simulink model "tractor_mu1109"  (R2022b)
settings: Solver=FixedStepDiscrete  StartTime=0.0  StopTime=20  FixedStep=0.001  RelTol=1e-3
model workspace (MAT data in the model file):
  P : object (value not decoded)
  w_2 : Simulink.Parameter (value not decoded)
undefined symbols (not defined in the file): A, a, B, b, C, D, DiscIntNeverNeededParam, Iz, K, k1, K1, k2, K2, L1, L2, m, magnitude, Phi, Sample_time, Steer_Ratio
libraries: simulink x26, slpidlib x13, Solver_SF x1, dsparch4 x1
(part 7 of 7)

== matlab function tractor_mu1109/软土扭矩分配/CBF-QP扭矩分配 ==
  data: dt_s input; selected_torques_n_m output; kappa input; dot_kappa input; kappa_valid input; input_gains input; previous_applied_torques_n_m input; nominal_torques_n_m input; base_torques_n_m input; wheel_limits_n_m input; front_steers_rad input; total_torque_n_m input; control_mz_n_m input; cbf_torque_upper_bounds output; cbf_active output; qp_status output; qp_objective output; disturbance_state_out output; disturbance_margins output
function [selected_torques_n_m, cbf_torque_upper_bounds, cbf_active, qp_status, qp_objective, disturbance_state_out, disturbance_margins] = MF_CBF_QP_TorqueAllocator(dt_s, kappa, dot_kappa, kappa_valid, input_gains, previous_applied_torques_n_m, nominal_torques_n_m, base_torques_n_m, wheel_limits_n_m, front_steers_rad, total_torque_n_m, control_mz_n_m)

% CBF-QP 安全扭矩分配模块
%
% 本模块完成：
% 1）滑移率动力学扰动估计；
% 2）CBF滑移安全扭矩上界计算；
% 3）考虑前轮转角的横摆力矩系数计算；
% 4）四轮扭矩QP优化分配。

persistent disturbance_state

if isempty(disturbance_state)
    disturbance_state = zeros(1, 4);
end

%% 输入整理

dt = max(double(dt_s), 0.0);

kappa_vec = row4_local(kappa);
dot_kappa_vec = row4_local(dot_kappa);
valid_vec = row4_local(kappa_valid);
gain_vec = row4_local(input_gains);
applied_vec = row4_local(previous_applied_torques_n_m);
nominal_vec = row4_local(nominal_torques_n_m);
base_vec = row4_local(base_torques_n_m);
limit_vec = row4_local(wheel_limits_n_m);

total_target = double(total_torque_n_m);
yaw_target = double(control_mz_n_m);

steer_input = double(front_steers_rad);

if numel(steer_input) >= 2
    delta_l = steer_input(1);
    delta_r = steer_input(2);
else
    delta_l = steer_input(1);
    delta_r = steer_input(1);
end

%% 轮端限幅整理

wheel_limits = zeros(1, 4);
base_torques = zeros(1, 4);
nominal_torques = zeros(1, 4);

for index = 1:4

    wheel_limits(index) = max(0.0, limit_vec(index));

    base_torques(index) = clamp_local(base_vec(index), 0.0, wheel_limits(index));

    nominal_torques(index) = clamp_local(nominal_vec(index), 0.0, wheel_limits(index));
end

%% 一、等效扰动估计

% 滑移率动力学：
% dot(kappa_i) = g_i * T_i + d_i
%
% 等效扰动估计：
% d_i = dot(kappa_i) - g_i * T_i

disturbance_margins = zeros(1, 4);
alpha_disturbance = first_order_alpha_local(dt, 0.15);

for index = 1:4

    gain = gain_vec(index);

    if valid_vec(index) > 0.5 && isfinite(gain)

        raw_estimate = dot_kappa_vec(index) - gain * applied_vec(index);

        disturbance_state(index) = disturbance_state(index) + ...
            alpha_disturbance * (raw_estimate - disturbance_state(index));

        residual = raw_estimate - disturbance_state(index);

    else

        residual = 0.0;
    end

    % 扰动估计不确定性裕度。
    disturbance_margins(index) = clamp_local(0.05 + 0.05 * abs(residual), 0.05, 5.0);
end

disturbance_state_out = disturbance_state;

%% 二、CBF滑移安全扭矩上界计算

% 安全函数：
% h_i = kappa_max - kappa_i
%
% CBF条件：
% dot(h_i) + gamma*h_i >= 0
%
% 由 dot(kappa_i) = g_i*T_i + d_i 可得：
% g_i*T_i + d_i + margin_i <= gamma*(kappa_max - kappa_i)
%
% 因此：
% T_i <= [gamma*(kappa_max-kappa_i) - d_i - margin_i] / g_i

kappa_max = 0.25;
cbf_gamma = 15.0;

cbf_torque_upper_bounds = zeros(1, 4);
cbf_active = zeros(1, 4);

for index = 1:4

    gain = gain_vec(index);

    if valid_vec(index) > 0.5 && isfinite(gain) && isfinite(kappa_vec(index))

        upper = (cbf_gamma * (kappa_max - kappa_vec(index)) ...
            - disturbance_state(index) ...
            - disturbance_margins(index)) / gain;

        if ~isfinite(upper)
            upper = wheel_limits(index);
        end

        upper = clamp_local(upper, 0.0, wheel_limits(index));

    else

        upper = wheel_limits(index);
    end

    cbf_torque_upper_bounds(index) = upper;

    % 若CBF上界低于基线扭矩，说明安全约束实际参与限幅。
    if upper < base_torques(index) - 1.0e-6
        cbf_active(index) = 1.0;
    end
end

%% 三、考虑前轮转角的横摆力矩映射系数

% 车辆几何参数。
lf = 2.043;
lr = 1.362;

track_front = 2.39;
track_rear = 2.33;

radius_front = 0.834;
radius_rear = 0.94;

% 当前QP只考虑轮端纵向驱动力产生的横摆力矩。
% 对前轮，驱动力方向随转角变化：
% F_x_body = F_i*cos(delta_i)
% F_y_body = F_i*sin(delta_i)
%
% 横摆力矩：
% M_z_i = x_i*F_y_body - y_i*F_x_body
%
% 因为 F_i = T_i/r_i，所以：
% yaw_coeff_i = (x_i*sin(delta_i) - y_i*cos(delta_i)) / r_i

yaw_coefficients = zeros(1, 4);

% 左前轮：x = lf, y = +track_front/2。
yaw_coefficients(1) = (lf * sin(delta_l) - 0.5 * track_front * cos(delta_l)) / radius_front;

% 右前轮：x = lf, y = -track_front/2。
yaw_coefficients(2) = (lf * sin(delta_r) + 0.5 * track_front * cos(delta_r)) / radius_front;

% 左后轮：x = -lr, y = +track_rear/2, delta = 0。
% 因为 sin(0)=0，所以 lr 项不直接进入纵向力横摆力矩。
yaw_coefficients(3) = -0.5 * track_rear / radius_rear;

% 右后轮：x = -lr, y = -track_rear/2, delta = 0。
yaw_coefficients(4) = 0.5 * track_rear / radius_rear;

%% 四、QP四轮扭矩优化分配

lower_bounds = zeros(1, 4);

[qp_torques, qp_status, qp_objective] = solve_torque_qp_local( ...
    nominal_torques, ...
    total_target, ...
    yaw_target, ...
    lower_bounds, ...
    cbf_torque_upper_bounds, ...
    yaw_coefficients);

%% 五、QP失败时安全降级

if qp_status > 0.5

    selected_torques_n_m = qp_torques;

else

    selected_torques_n_m = zeros(1, 4);

    for index = 1:4
        selected_torques_n_m(index) = clamp_local(base_torques(index), 0.0, cbf_torque_upper_bounds(index));
    end
end

end


function [solution, status, objective] = solve_torque_qp_local(nominal, total_target, yaw_target, lower, upper, yaw)

% 四轮扭矩边界约束QP求解器
%
% 决策变量：
% T = [T1, T2, T3, T4]
%
% 目标函数：
% J = 0.5*w_nominal*sum((T_i - T_nom_i)^2)
%   + 0.5*w_total*(sum(T_i) - T_total_ref)^2
%   + 0.5*w_yaw*(yaw*T' - Mz_ref)^2
%   + regularization*sum(T_i^2)
%
% 约束：
% lower_i <= T_i <= upper_i
%
% 由于只有4个决策变量，这里采用主动集枚举方法，
% 每个变量枚举为下界、自由、上界三种状态。

status = -1.0;
objective = NaN;
solution = zeros(1, 4);

%% 可行性预检查

for index = 1:4
    if upper(index) < lower(index) || ~isfinite(upper(index)) || ~isfinite(lower(index))
        return;
    end
end

%% 权重参数

weight_nominal = 1.0;
weight_total = 1.12;
weight_yaw = 0.02;
regularization = 1.0e-6;

%% 构造二次型矩阵和线性项

H = zeros(4, 4);
linear = zeros(1, 4);

for row = 1:4

    for col = 1:4

        % 总扭矩项对 Hessian 的贡献。
        % 横摆力矩项对 Hessian 的贡献。
        H(row, col) = H(row, col) + weight_total + weight_yaw * yaw(row) * yaw(col);
    end

    % 名义扭矩跟踪项和正则化项。
    H(row, row) = H(row, row) + weight_nominal + 2.0 * regularization;

    % 线性项。
    linear(row) = linear(row) ...
        - weight_nominal * nominal(row) ...
        - weight_total * total_target ...
        - weight_yaw * yaw_target * yaw(row);
end

%% 主动集枚举

best_objective = Inf;

% -1：固定在下界；
%  0：自由变量；
%  1：固定在上界。
states = [-1.0, 0.0, 1.0];

for i1 = 1:3
    for i2 = 1:3
        for i3 = 1:3
            for i4 = 1:3

                activity = [states(i1), states(i2), states(i3), states(i4)];

                candidate = zeros(1, 4);
                free_indices = zeros(1, 4);
                nfree = 0;

                %% 设置固定变量并记录自由变量

                for index = 1:4

                    if activity(index) < -0.5

                        candidate(index) = lower(index);

                    elseif activity(index) > 0.5

                        candidate(index) = upper(index);

                    else

                        nfree = nfree + 1;
                        free_indices(nfree) = index;
                    end
                end

                %% 求解自由变量

                if nfree > 0

                    A = zeros(4, 4);
                    b = zeros(1, 4);

                    for rr = 1:nfree

                        row = free_indices(rr);
                        fixed_contribution = 0.0;

                        for col = 1:4
                            if activity(col) ~= 0.0
                                fixed_contribution = fixed_contribution + H(row, col) * candidate(col);
                            end
                        end

                        b(rr) = -linear(row) - fixed_contribution;

                        for cc = 1:nfree
                            A(rr, cc) = H(row, free_indices(cc));
                        end
                    end

                    [free_solution, ok] = solve_linear_system4_local(A, b, nfree);

                    if ok <= 0.5
                        continue;
                    end

                    for rr = 1:nfree
                        candidate(free_indices(rr)) = free_solution(rr);
                    end
                end

                %% 可行性检查

                feasible = 1.0;

                for index = 1:4

                    if candidate(index) < lower(index) - 1.0e-7 || ...
                            candidate(index) > upper(index) + 1.0e-7 || ...
                            ~isfinite(candidate(index))

                        feasible = 0.0;
                    end

                    candidate(index) = clamp_local(candidate(index), lower(index), upper(index));
                end

                if feasible <= 0.5
                    continue;
                end

                %% 计算目标函数

                obj = quadratic_objective_local(candidate, H, linear);

                if obj < best_objective

                    best_objective = obj;
                    solution = candidate;
                    status = 1.0;
                    objective = obj;
                end
            end
        end
    end
end

end


function [x, ok] = solve_linear_system4_local(A, b, n)

% 求解最多4维线性方程组 A*x=b。
% 采用带部分主元选择的高斯消元法。

x = zeros(1, 4);
ok = 1.0;

if n == 0
    return;
end

aug = zeros(4, 5);

for row = 1:n

    for col = 1:n
        aug(row, col) = A(row, col);
    end

    aug(row, n + 1) = b(row);
end

%% 前向消元

for col = 1:n

    pivot_row = col;
    pivot_abs = abs(aug(col, col));

    for row = col:n
        if abs(aug(row, col)) > pivot_abs
            pivot_abs = abs(aug(row, col));
            pivot_row = row;
        end
    end

    if pivot_abs <= 1.0e-12 || ~isfinite(pivot_abs)
        ok = 0.0;
        return;
    end

    if pivot_row ~= col

        temp = aug(col, :);
        aug(col, :) = aug(pivot_row, :);
        aug(pivot_row, :) = temp;
    end

    for row = col + 1:n

        factor = aug(row, col) / aug(col, col);

        if factor ~= 0.0

            for entry = col:n + 1
                aug(row, entry) = aug(row, entry) - factor * aug(col, entry);
            end
        end
    end
end

%% 回代

for row = n:-1:1

    residual = aug(row, n + 1);

    for col = row + 1:n
        residual = residual - aug(row, col) * x(col);
    end

    pivot = aug(row, row);

    if abs(pivot) <= 1.0e-12
        ok = 0.0;
        return;
    end

    x(row) = residual / pivot;

    if ~isfinite(x(row))
        ok = 0.0;
        return;
    end
end

end


function value = quadratic_objective_local(torques, H, linear)

% QP目标函数：
% J = 0.5*T*H*T' + linear*T'

value = 0.0;

for row = 1:4

    for col = 1:4
        value = value + 0.5 * torques(row) * H(row, col) * torques(col);
    end

    value = value + linear(row) * torques(row);
end

end


function output = row4_local(values)

% 将输入信号整理为 1×4 行向量。

input_values = double(values);
output = zeros(1, 4);

for index = 1:4
    output(index) = input_values(index);
end

end


function alpha = first_order_alpha_local(dt, time_constant_s)

% 一阶低通滤波系数。

if dt <= 0.0 || time_constant_s <= 0.0
    alpha = 1.0;
else
    alpha = dt / (time_constant_s + dt);
end

end


function value = clamp_local(value_in, lower, upper)

% 数值限幅函数。

value = min(max(double(value_in), double(lower)), double(upper));

end

== matlab function tractor_mu1109/软土扭矩分配/牵引效率评价计算 ==
  data: dt_s input; eta_wg_E output; drawbar_power_w input; wheel_power_w input; E_wg output; E_w output; drawbar_force input
function [eta_wg_E, E_wg, E_w] = MF_EnergyWeightedTractionEfficiency(dt_s, drawbar_power_w, wheel_power_w, drawbar_force)

persistent E_wg_state E_w_state

if isempty(E_wg_state)
    E_wg_state = 0.0;
    E_w_state = 0.0;
end

dt = max(double(dt_s), 0.0);

epsilon_E = 1.0;   % 防止低能量窗口除零，可根据功率量级调整

%window_enable = wheel_power_w > 100 && drawbar_force > 10;
window_enable = 1;

if double(window_enable) > 0.5
    E_wg_state = E_wg_state + max(0.0, double(drawbar_power_w)) * dt;
    E_w_state = E_w_state + max(0.0, double(wheel_power_w)) * dt;
end

eta_wg_E = E_wg_state / (E_w_state + epsilon_E);

E_wg = E_wg_state;
E_w = E_w_state;

end

== matlab function tractor_mu1109/驱动防滑模块/起步探测 ==
  data: v_ref output size=[4 1]; dv output size=[4 1]; spin_on_raw output boolean size=[4 1]; spin_clear_raw output boolean size=[4 1]; no_move_raw output boolean; w input size=[4 1]; vx input; vy input; ax input; r input; delta input size=[4 1]; speed_src_valid input; T_actual input size=[4 1]; T_max input size=[4 1]; reset input; move_ok output boolean; speed_on_raw output boolean; speed_off_raw output boolean; consistency_ok output boolean; source_immediate_bad output boolean; drive_active output boolean; diag_motion output size=[4 1]; P parameter
function [v_ref, dv, spin_on_raw, spin_clear_raw, no_move_raw, move_ok, ...
          speed_on_raw, speed_off_raw, consistency_ok, ...
          source_immediate_bad, drive_active, diag_motion] = ...
    LaunchTCS_Motion(w, vx, vy, ax, r, delta, speed_src_valid, ...
                     T_actual, T_max, reset, P)
%#codegen
% 前级：只计算运动量和瞬时判据，不做计时、不锁存、不决定 stage。
% 四轮顺序 [FL;FR;RL;RR]。

persistent initialized w_f vx_f vy_f ax_f r_f vx_prev dv_prev

if isempty(initialized)
    initialized = false;
    w_f = zeros(4,1); vx_f = 0; vy_f = 0; ax_f = 0; r_f = 0;
    vx_prev = 0; dv_prev = zeros(4,1);
end

%% 1. 先统一定义所有局部变量（避免"未定义"报错）
w_s = zeros(4,1);
delta_s = zeros(4,1);
vx_s = 0; vy_s = 0; ax_s = 0; r_s = 0;
raw_ok = true;
vx_dot = 0;
v_ref = zeros(4,1);
dv = zeros(4,1);
wheel_speed = zeros(4,1);
dv_rate = zeros(4,1);
active = zeros(4,1);

%% 2. 输入检查：异常值用上一拍滤波值顶替，并记录故障
for i = 1:4
    w_s(i) = w(i);
    delta_s(i) = delta(i);
    if isnan(w_s(i)) || isinf(w_s(i))
        w_s(i) = w_f(i); raw_ok = false;
    end
    if isnan(delta_s(i)) || isinf(delta_s(i))
        delta_s(i) = 0; raw_ok = false;
    end
end

vx_s = vx; vy_s = vy; ax_s = ax; r_s = r;
if isnan(vx_s) || isinf(vx_s), vx_s = vx_f; raw_ok = false; end
if isnan(vy_s) || isinf(vy_s), vy_s = vy_f; raw_ok = false; end
if isnan(ax_s) || isinf(ax_s), ax_s = ax_f; raw_ok = false; end
if isnan(r_s)  || isinf(r_s),  r_s  = r_f;  raw_ok = false; end

src_flag_ok = ~(isnan(speed_src_valid) || isinf(speed_src_valid));
src_val = speed_src_valid;
if ~src_flag_ok, src_val = 0; end

%% 3. 滤波与车速微分
do_init = (reset > 0.5) || ~initialized;
if do_init
    initialized = true;
    w_f = w_s; vx_f = vx_s; vy_f = vy_s; ax_f = ax_s; r_f = r_s;
    vx_prev = vx_f;
    dv_prev = zeros(4,1);
else
    vx_prev = vx_f;
    w_f  = (1-P.alpha_w)  * w_f  + P.alpha_w  * w_s;
    vx_f = (1-P.alpha_v)  * vx_f + P.alpha_v  * vx_s;
    vy_f = (1-P.alpha_vy) * vy_f + P.alpha_vy * vy_s;
    ax_f = (1-P.alpha_a)  * ax_f + P.alpha_a  * ax_s;
    r_f  = (1-P.alpha_r)  * r_f  + P.alpha_r  * r_s;
end
vx_dot = (vx_f - vx_prev) / P.Ts;

%% 4. 四轮参考速度与轮端-车体速度差
for i = 1:4
    v_ref(i) = max(0, (vx_f - r_f*P.y(i))*cos(delta_s(i)) ...
                     + (vy_f + r_f*P.x(i))*sin(delta_s(i)));
    wheel_speed(i) = max(w_f(i), 0) * P.R(i);
    dv(i) = wheel_speed(i) - v_ref(i);
    if do_init
        dv_rate(i) = 0;
    else
        dv_rate(i) = (dv(i) - dv_prev(i)) / P.Ts;
    end
end

%% 5. 信号健康与有效驱动
plausible = (vx_f >= P.vx_min) && (vx_f <= P.vx_max);
src_ok = (src_val > 0.5) && src_flag_ok;
actual_ok = true;

for i = 1:4
    cap_valid = ~(isnan(T_max(i)) || isinf(T_max(i))) && ...
                (T_max(i) >= P.TcapFloor(i));
    act_valid = ~(isnan(T_actual(i)) || isinf(T_actual(i)));
    if ~act_valid, actual_ok = false; end
    if cap_valid && act_valid
        active(i) = double(T_actual(i) >= P.applied_active_frac * T_max(i));
    end
end

drive_active = any(active > 0.5);
source_immediate_bad = (~raw_ok) || (~src_ok) || (~plausible) || ...
                       (~actual_ok);
consistency_ok = (~source_immediate_bad) && ...
                 (abs(vx_dot - ax_f) <= P.a_cons_max);

%% 6. 四轮空转瞬时条件
spin_on_raw = false(4,1);
spin_clear_raw = false(4,1);
for i = 1:4
    spin_on_raw(i) = (~source_immediate_bad) && ...
        (dv(i) > P.dv_spin_on) && ...
        (wheel_speed(i) > P.v_wheel_min) && ...
        (active(i) > 0.5) && ...
        ((ax_f < P.a_spin_max) || (dv_rate(i) > P.dv_growth_on));
    spin_clear_raw(i) = (~source_immediate_bad) && (dv(i) < P.dv_spin_off);
end

%% 7. 未起动与车速切换瞬时条件
no_move_raw = (~source_immediate_bad) && drive_active && ...
              (vx_f < P.v_move_on) && (ax_f < P.a_response);
move_ok = (~source_immediate_bad) && ...
          ((vx_f >= P.v_move_on) || (ax_f >= P.a_response));
speed_on_raw = (~source_immediate_bad) && consistency_ok && ...
               (vx_f >= P.v_valid_on);
speed_off_raw = source_immediate_bad || (vx_f < P.v_valid_off);

%% 8. 观察量与历史更新
diag_motion = [vx_f; ax_f; vx_dot; max(dv)];
dv_prev = dv;

end

== matlab function tractor_mu1109/驱动防滑模块/起步扭矩控制 ==
  data: stage input uint8; T_pref output size=[4 1]; spin_mask input boolean size=[4 1]; T_base input size=[4 1]; T_max input size=[4 1]; reset input; T_lim_out output size=[4 1]; T_cmd output size=[4 1]; diag_torque output size=[4 1]; P parameter
function [T_pref, T_lim_out, T_cmd, diag_torque] = LaunchTCS_Torque(stage, spin_mask, T_base, T_max, reset, P)
%--------------------------------------------------------------------------
% 函数名称：LaunchTCS_Torque
%
% 职责：
%   执行 Stateflow 已经判定好的状态所对应的扭矩动作，输出
%   偏好扭矩 T_pref、逐轮运行上界 T_lim_out 和实际命令扭矩 T_cmd。
%
% 本函数不做的事：
%   不判断应进入哪个状态、不累计确认时间、不锁存空转或车速可信。
%   stage 与 spin_mask 均由 launch_state 状态机输入，
%   避免模型中出现第二套状态机。
%
% 四轮顺序：1=FL，2=FR，3=RL，4=RR；扭矩单位 N·m。
%
% 输入：
%   stage      uint8，状态编号
%              0 起步探测  1 正常起步  2 重载未起动  3 单轮空转
%              4 多轮空转  5 作业阶段  6 信号保护   255 未使能
%   spin_mask  4×1 逻辑量，状态机锁存后的四轮空转标志
%   T_base     4×1，基础四轮扭矩需求，N·m
%   T_max      4×1，当前轮端能力上限，N·m
%   reset      标量，复位信号
%   P          参数结构体
%
% 输出：
%   T_pref      4×1，当前状态下的四轮偏好扭矩
%   T_lim_out   4×1，四轮运行扭矩上界
%   T_cmd       4×1，本拍实际下发的四轮扭矩
%   diag_torque 4×1，观察量
%
% 接口说明：
%   T_pref 与 T_lim_out 也是后续统一扭矩分配器的接口量，
%   前者作为偏好目标，后者作为逐轮不等式约束。
%   运行上界属于算法设定的控制边界，不是已辨识出的轮胎附着极限 [2]
%--------------------------------------------------------------------------

%#codegen

% 持久变量，仅用于扭矩的渐变过程，不参与状态判定：
%   initialized ：首次调用标志
%   q           ：起步扭矩探测比例
%   total_scale ：多轮空转时的总扭矩比例
%   Tlim        ：四轮动态运行上界
%   Tcmd_prev   ：上一拍命令扭矩，用于变化率限制
%   prev_stage  ：上一拍状态，用于识别重新回到起步探测
persistent initialized q total_scale Tlim Tcmd_prev prev_stage

% cap ：本拍可用的四轮能力上限
% base：本拍整理后的四轮基础扭矩需求
cap=zeros(4,1); base=zeros(4,1);
for i=1:4
% 能力上限有效（非 NaN/Inf 且不低于地板值）时采用该值；
% 无效时该轮能力按 0 处理，即本拍不允许该轮输出驱动扭矩，
% 不用未经核实的默认峰值顶替。
if ~(isnan(T_max(i))||isinf(T_max(i))) && T_max(i)>=P.TcapFloor(i), cap(i)=T_max(i); else, cap(i)=0; end
% 基础扭矩只取正向部分，本版不处理倒车与制动；
% 若该轮基础扭矩无效，则保持预置的 0。
if ~(isnan(T_base(i))||isinf(T_base(i))), base(i)=max(T_base(i),0); end
end

% 首次调用初始化：
% 从最小探测比例起步，运行上界初值取当前能力，命令扭矩为 0，
% prev_stage 置 255，使首次进入起步探测时不触发"从作业阶段回落"的重置。
if isempty(initialized)
    initialized=true; q=P.q_start; total_scale=1; Tlim=cap; Tcmd_prev=zeros(4,1); prev_stage=uint8(255);
end

% 输出预置，保证所有分支（含提前 return）都有确定的维度和初值。
T_pref=zeros(4,1); T_lim_out=zeros(4,1); T_cmd=zeros(4,1); diag_torque=zeros(4,1);

% 复位或未使能（stage=255）：
% 清空全部渐变记忆；T_lim_out 输出当前能力值，表示上界未被收紧；
% 但 T_cmd 仍为预置的 0，因此本拍不产生驱动。
% 注意此分支直接 return，diag_torque 保持全 0。
if reset>0.5 || stage==uint8(255)
    q=P.q_start; total_scale=1; Tlim=cap; Tcmd_prev=zeros(4,1); prev_stage=stage; T_lim_out=cap; return;
end

% 防御性处理：若状态机给出 7~254 的未定义编码，一律按保护状态（6）执行。
s=stage; if s>uint8(6), s=uint8(6); end

% 从作业阶段重新回落到静止起步探测时，探测比例重新从最小值开始，
% 避免带着 q=1 直接施加大扭矩而诱发空转。
if s==uint8(0)&&prev_stage==uint8(5), q=P.q_start; end

% 状态 0/1：起步探测与正常起步。
% 探测比例按 q_probe_rate 逐步放开，上限为 1；
% 偏好扭矩取"基础需求"与"当前允许比例对应扭矩"的较小值。
if s==uint8(0)||s==uint8(1)
    q=min(1,q+P.q_probe_rate*P.Ts);
for i=1:4, T_pref(i)=min(base(i),q*cap(i)); end

% 状态 2：重载未起动。
% 车体未动但尚未确认空转，只允许缓慢探测，
% 且探测比例的上限收紧为 q_no_move_max。
elseif s==uint8(2)
    q=min(P.q_no_move_max,q+P.q_no_move_rate*P.Ts);
for i=1:4, T_pref(i)=min(base(i),q*cap(i)); end

% 状态 3：单轮空转。
% 探测比例回退；偏好扭矩仍以基础扭矩为准，
% 实际限扭通过下面的 Tlim 与最终的 target=min(T_pref,T_lim_out) 实现 [3]
elseif s==uint8(3)
    q=max(P.q_start,q-P.q_spin_down*P.Ts); T_pref=base;
for i=1:4
% 空转轮按 q_limit_cut_rate 收紧运行上界，但不低于 q_limit_floor*cap；
% 其余车轮按 q_limit_rec_rate 缓慢恢复上界。
% 这里不把被收掉的扭矩主动转移给其他车轮，以免诱发多轮空转 [3]
if spin_mask(i), Tlim(i)=max(P.q_limit_floor*cap(i),Tlim(i)-P.q_limit_cut_rate*cap(i)*P.Ts); else, Tlim(i)=min(cap(i),Tlim(i)+P.q_limit_rec_rate*cap(i)*P.Ts); end
end

% 状态 4：多轮空转。
% 不再逐轮处理，而是整体回退总驱动需求：
% total_scale 按 q_multi_cut_rate 下降至不低于 q_multi_min，
% 偏好扭矩按该比例整体缩放，同时收紧全部车轮的运行上界 [3]
elseif s==uint8(4)
    q=max(P.q_start,q-P.q_spin_down*P.Ts); total_scale=max(P.q_multi_min,total_scale-P.q_multi_cut_rate*P.Ts); T_pref=total_scale*base;
for i=1:4, Tlim(i)=max(P.q_limit_floor*cap(i),Tlim(i)-P.q_limit_cut_rate*cap(i)*P.Ts); end

% 状态 5：作业阶段接口。
% 当前版本把基础扭矩直通为偏好扭矩；
% 后续替换为作业过程滑转控制的输出（滑转率计算、目标滑转率、
% 四轮滑转跟踪扭矩）[3]
elseif s==uint8(5)
    q=1; T_pref=base;

% 状态 6：信号保护。
% 关键信号不可信时快速回退探测比例，
% 并把偏好扭矩压到 q_protect 对应的较小比例以内。
else
    q=max(P.q_start,q-P.q_protect_down*P.Ts);
for i=1:4, T_pref(i)=min(base(i),P.q_protect*cap(i)); end
end

% 只要不处于多轮空转状态，总扭矩比例就按 q_multi_rec_rate 回升至 1。
if s~=uint8(4), total_scale=min(1,total_scale+P.q_multi_rec_rate*P.Ts); end

% 既非单轮空转也非多轮空转时，四轮运行上界统一缓慢恢复。
% 单轮空转与多轮空转分支已在上面各自处理过 Tlim，这里不重复更新。
% 由此可知：进入作业阶段后，先前收紧的上界也是渐进恢复，不会瞬间解除。
if s~=uint8(3)&&s~=uint8(4)
for i=1:4, Tlim(i)=min(cap(i),Tlim(i)+P.q_limit_rec_rate*cap(i)*P.Ts); end
end

% 把运行上界与偏好扭矩都夹到 [0, cap] 区间。
% 其中 min(·,cap(i)) 还保证了实时能力下降时，运行上界立即跟随下降 [3]
for i=1:4, Tlim(i)=min(max(Tlim(i),0),cap(i)); T_pref(i)=min(max(T_pref(i),0),cap(i)); end

% 对外输出的运行上界默认等于内部 Tlim。
T_lim_out=Tlim;

% 多轮空转时再叠加总体比例限制；保护状态时再叠加保护比例限制。
% 这两行是向量运算，一次处理四个车轮。
if s==uint8(4), T_lim_out=min(T_lim_out,total_scale*cap); elseif s==uint8(6), T_lim_out=min(T_lim_out,P.q_protect*cap); end

for i=1:4
% target：本轮本拍的目标扭矩，同时满足偏好扭矩与运行上界。
% rise/fall：按能力比例折算出的单拍最大上升量与下降量，
% 下降速率通常设得比上升快，便于发生空转时及时降扭 [3]
    target=min(T_pref(i),T_lim_out(i)); rise=P.cmd_rise_rate*cap(i)*P.Ts; fall=P.cmd_fall_rate*cap(i)*P.Ts;
% 目标高于上一拍则按上升速率逼近；低于上一拍则按下降速率逼近。
if target>=Tcmd_prev(i), T_cmd(i)=min(target,Tcmd_prev(i)+rise); else, T_cmd(i)=max(target,Tcmd_prev(i)-fall); end
% 变化率限制之后再做一次硬夹取：
% 保证 0 <= T_cmd(i) <= T_lim_out(i)。
% 这一步使运行上界优先于下降变化率，上界突然收紧时命令扭矩可立即降入上界以内。
    T_cmd(i)=min(max(T_cmd(i),0),T_lim_out(i));
end

% 更新历史量：本拍命令扭矩与本拍状态，供下一拍使用。
% diag_torque = [探测比例 q；总扭矩比例 total_scale；
%                当前空转轮数量；当前状态编号]
Tcmd_prev=T_cmd; prev_stage=s; diag_torque=[q;total_scale;sum(double(spin_mask));double(s)];
end

== stateflow chart tractor_mu1109/驱动防滑模块/launch_state ==
  settings: updateMethod=DISCRETE  sampleTime=0.001
  state MONITOR [parallel]
    entry:
    spin_on_t=zeros(4,1); spin_clear_t=zeros(4,1); spin_mask=false(4,1); nspin=0; no_move_t=0;
    no_move_confirmed=false; speed_on_t=0; speed_off_t=0; speed_valid=false; cons_bad_t=0;
    source_bad=false; desired_stage=uint8(255);
    during:
    if enable<=0.5 || reset>0.5
    spin_on_t=zeros(4,1); spin_clear_t=zeros(4,1); spin_mask=false(4,1); nspin=0; no_move_t=0;
    no_move_confirmed=false; speed_on_t=0; speed_off_t=0; speed_valid=false; cons_bad_t=0;
    source_bad=false; if enable<=0.5, desired_stage=uint8(255); else, desired_stage=uint8(0);
    end
    else
    for i=1:4
    if spin_on_raw(i), spin_on_t(i)=min(P.t_spin_on,spin_on_t(i)+P.Ts); spin_clear_t(i)=0;
    else, spin_on_t(i)=max(0,spin_on_t(i)-P.Ts); if spin_clear_raw(i), spin_clear_t(i)=min(P.t_spin_clear,spin_clear_t(i)+P.Ts);
    else, spin_clear_t(i)=0;
    end, end
    if spin_on_t(i)>=P.t_spin_on, spin_mask(i)=true; end
    if spin_clear_t(i)>=P.t_spin_clear, spin_mask(i)=false; end
    end
    nspin=sum(double(spin_mask));
    if no_move_raw, no_move_t=min(P.t_no_move,no_move_t+P.Ts); elseif move_ok, no_move_t=0; else, no_move_t=max(0,no_move_t-P.Ts); end
    no_move_confirmed=no_move_t>=P.t_no_move;
    if consistency_ok, cons_bad_t=max(0,cons_bad_t-P.Ts); else, cons_bad_t=min(P.t_cons_bad,cons_bad_t+P.Ts); end
    source_bad=source_immediate_bad || cons_bad_t>=P.t_cons_bad;
    if ~speed_valid
    if speed_on_raw && nspin<=1 && ~source_bad, speed_on_t=min(P.t_speed_on,speed_on_t+P.Ts); else, speed_on_t=0; end
    if speed_on_t>=P.t_speed_on, speed_valid=true; speed_off_t=0; end
    else
    if speed_off_raw || nspin>=2 || source_bad, speed_off_t=min(P.t_speed_off,speed_off_t+P.Ts); else, speed_off_t=0; end
    if speed_off_t>=P.t_speed_off, speed_valid=false; speed_on_t=0; end
    end
    if source_bad, desired_stage=uint8(6); elseif nspin>=2, desired_stage=uint8(4);
    elseif nspin==1, desired_stage=uint8(3); elseif speed_valid, desired_stage=uint8(5);
    elseif no_move_confirmed, desired_stage=uint8(2); elseif move_ok, desired_stage=uint8(1);
    else, desired_stage=uint8(0); end
    end
    settings: executionOrder=1
  state MODE [parallel]
    settings: executionOrder=2
    state DISABLED
      entry: stage = uint8(255);
    state START_PROBE
      entry: stage = uint8(0);
    state NORMAL_LAUNCH
      entry: stage = uint8(1);
    state HEAVY_NO_MOVE
      entry: stage = uint8(2);
    state SINGLE_SPIN
      entry: stage = uint8(3);
    state MULTI_SPIN
      entry: stage = uint8(4);
    state WORK_PASS
      entry: stage = uint8(5);
    state PROTECT
      entry: stage = uint8(6);
    (default) -> DISABLED
    (junction 98) -> START_PROBE [order 2] : [desired_stage == uint8(0)]
    (junction 98) -> DISABLED [order 1] : [desired_stage == uint8(255)]
    DISABLED -> (junction 98) : [desired_stage ~= uint8(255)]
    START_PROBE -> (junction 98) : [desired_stage ~= uint8(0)]
    (junction 98) -> HEAVY_NO_MOVE [order 4] : [desired_stage == uint8(2)]
    (junction 98) -> NORMAL_LAUNCH [order 3] : [desired_stage == uint8(1)]
    HEAVY_NO_MOVE -> (junction 98) : [desired_stage ~= uint8(2)]
    NORMAL_LAUNCH -> (junction 98) : [desired_stage ~= uint8(1)]
    (junction 98) -> MULTI_SPIN [order 6] : [desired_stage == uint8(4)]
    (junction 98) -> SINGLE_SPIN [order 5] : [desired_stage == uint8(3)]
    MULTI_SPIN -> (junction 98) : [desired_stage ~= uint8(4) && after(0.2,sec)]
    SINGLE_SPIN -> (junction 98) : [desired_stage ~= uint8(3) && after(0.2,sec)]
    (junction 98) -> PROTECT [order 8] : [desired_stage == uint8(6)]
    PROTECT -> (junction 98) : [desired_stage ~= uint8(6)]
    (junction 98) -> WORK_PASS [order 7] : [desired_stage == uint8(5)]
    WORK_PASS -> (junction 98) : [desired_stage ~= uint8(5)]
  data: spin_on_raw input boolean size=[4 1]; spin_clear_raw input boolean size=[4 1]; no_move_raw input boolean size=1; move_ok input boolean size=1; speed_on_raw input boolean size=1; speed_off_raw input boolean size=1; consistency_ok input boolean size=1; source_immediate_bad input boolean size=1; enable input double size=1; reset input double size=1; stage output uint8; spin_mask output boolean size=[4 1]; speed_valid output boolean; no_move_confirmed output boolean; source_bad output boolean; nspin output double; P parameter; spin_on_t local size=[4 1]; spin_clear_t local size=[4 1]; no_move_t local; speed_on_t local; speed_off_t local; cons_bad_t local; desired_stage local uint8; i local double size=1
